simulink model "rfsoc4x2_ospfb_128"  (R2021a)
settings: Solver=VariableStepAuto  StartTime=0.0  StopTime=2048  RelTol=1e-3
undefined symbols (not defined in the file): pfb_coeff_gen_calc
libraries: xbsIndex_r4 x37092, casper_library_delays x737, casper_library_misc x68, xps_library x1
(part 120 of 339)

== system rfsoc4x2_ospfb_128/pfb_fir_real8/pol1_in9_last_tap ==
  din : Inport
  sync : Inport  Port=2
  coeff : Inport  Port=3
  Delay : xbsIndex_r4/Delay  rst=off  infoeditControl=Selection of Reset will increase slice count due to use of real FFs and instead of SRLs  en=off  latency=mult_latency  reg_retiming=off  dbl_ovrd=off  block_type=delay
      settings: xl_area=[0, 0, 0, 0, 0, 0, 0]  block_version=9.1.01
  Mult : xbsIndex_r4/Mult  precision=Full  arith_type="Signed  (2's comp)"  n_bits=8  bin_pt=2  quantization=Truncate  overflow=Wrap  en=off  latency=mult_latency  use_behavioral_HDL=on  opt=Speed  use_embedded=off  optimum_pipeline=off  pipeline=on  dbl_ovrd=off  use_rpm=on  placement_style=Rectangular shape  block_type=mult
      settings: infoedit=Hardware notes: To use the internal pipeline stage of the dedicated multiplier you must select 'Pipeline for maximum performance'.  xl_area=[0, 0, 0, 0, 0, 0, 0]  block_version=9.1.01
  Reinterpret : xbsIndex_r4/Reinterpret  force_arith_type=on  arith_type="Signed  (2's comp)"  force_bin_pt=on  bin_pt=CoeffBitWidth - 1  block_type=reinterpret
      settings: infoedit="Changes signal type without altering the binary representation.   You can changed the signal between signed and unsigned, and relocate the binary point.<P><P>Hardware notes: In hardware this block costs nothing.<P><P>Example:  Suppose the input is 6 bits wide, signed, with 2 fractional bits, and the output is forced to unsigned with 0 fractional bits.  Then an input of -2.0 (1110.00 in binary 2's complement) becomes an output of 56 (111000 in binary)."  block_version=9.1.01
  Reinterpret1 : xbsIndex_r4/Reinterpret  force_arith_type=on  arith_type="Signed  (2's comp)"  force_bin_pt=on  bin_pt=BitWidthIn - 1  block_type=reinterpret
      settings: infoedit="Changes signal type without altering the binary representation.   You can changed the signal between signed and unsigned, and relocate the binary point.<P><P>Hardware notes: In hardware this block costs nothing.<P><P>Example:  Suppose the input is 6 bits wide, signed, with 2 fractional bits, and the output is forced to unsigned with 0 fractional bits.  Then an input of -2.0 (1110.00 in binary 2's complement) becomes an output of 56 (111000 in binary)."  block_version=9.1.01
  tap_out : Outport  VectorParamsAs1DForOutWhenUnconnected=off
  sync_out : Outport  Port=2  VectorParamsAs1DForOutWhenUnconnected=off
  wires:
  Delay/1 -> sync_out/1
  din/1 -> Reinterpret1/1
  sync/1 -> Delay/1
  coeff/1 -> Reinterpret/1
  Reinterpret/1 -> Mult/2
  Mult/1 -> tap_out/1
  Reinterpret1/1 -> Mult/1

== system rfsoc4x2_ospfb_128/pfb_fir_real8/pol1_in9_tap2 ==
  din : Inport
  sync : Inport  Port=2
  coeff : Inport  Port=3
  Mult : xbsIndex_r4/Mult  precision=Full  arith_type="Signed  (2's comp)"  n_bits=8  bin_pt=2  quantization=Truncate  overflow=Wrap  en=off  latency=mult_latency  use_behavioral_HDL=on  opt=Speed  use_embedded=off  optimum_pipeline=off  pipeline=on  dbl_ovrd=off  use_rpm=on  placement_style=Rectangular shape  block_type=mult
      settings: infoedit=Hardware notes: To use the internal pipeline stage of the dedicated multiplier you must select 'Pipeline for maximum performance'.  xl_area=[0, 0, 0, 0, 0, 0, 0]  block_version=9.1.01
  Reinterpret : xbsIndex_r4/Reinterpret  force_arith_type=on  arith_type="Signed  (2's comp)"  force_bin_pt=on  bin_pt=coeff_frac_width  block_type=reinterpret
      settings: infoedit="Changes signal type without altering the binary representation.   You can changed the signal between signed and unsigned, and relocate the binary point.<P><P>Hardware notes: In hardware this block costs nothing.<P><P>Example:  Suppose the input is 6 bits wide, signed, with 2 fractional bits, and the output is forced to unsigned with 0 fractional bits.  Then an input of -2.0 (1110.00 in binary 2's complement) becomes an output of 56 (111000 in binary)."  block_version=9.1.01
  Reinterpret1 : xbsIndex_r4/Reinterpret  force_arith_type=on  arith_type="Signed  (2's comp)"  force_bin_pt=on  bin_pt=data_width - 1  block_type=reinterpret
      settings: infoedit="Changes signal type without altering the binary representation.   You can changed the signal between signed and unsigned, and relocate the binary point.<P><P>Hardware notes: In hardware this block costs nothing.<P><P>Example:  Suppose the input is 6 bits wide, signed, with 2 fractional bits, and the output is forced to unsigned with 0 fractional bits.  Then an input of -2.0 (1110.00 in binary 2's complement) becomes an output of 56 (111000 in binary)."  block_version=9.1.01
  Slice : xbsIndex_r4/Slice  nbits=coeff_width  boolean_output=off  mode=Lower Bit Location + Width  bit1=0  base1=MSB of Input  bit0=0  base0=LSB of Input  dbl_ovrd=off  block_type=slice
      settings: infoedit="Extracts a given range of bits from each input sample and presents it at the output.  The output type is ordinarily unsigned with binary point at zero, but can be Boolean when the slice is one bit wide.<P><P>Hardware notes: In hardware this block costs nothing."  block_version=9.1.01
  Slice1 : xbsIndex_r4/Slice  nbits=0  boolean_output=off  mode=Two Bit Locations  bit1=0  base1=MSB of Input  bit0=coeff_width  base0=LSB of Input  dbl_ovrd=off  block_type=slice
      settings: infoedit="Extracts a given range of bits from each input sample and presents it at the output.  The output type is ordinarily unsigned with binary point at zero, but can be Boolean when the slice is one bit wide.<P><P>Hardware notes: In hardware this block costs nothing."  block_version=9.1.01
  delay_bram : casper_library_delays/delay_bram  DelayLen=delay  bram_latency=bram_latency  use_dsp48=off  async=off
      settings: SourceProductName=CASPER DSP Blockset
  sync_delay : casper_library_delays/sync_delay  DelayLen=delay
      settings: SourceProductName=CASPER DSP Blockset
  dout : Outport  VectorParamsAs1DForOutWhenUnconnected=off
  sync_out : Outport  Port=2  VectorParamsAs1DForOutWhenUnconnected=off
  coeff_out : Outport  Port=3  VectorParamsAs1DForOutWhenUnconnected=off
  taps_out : Outport  Port=4  VectorParamsAs1DForOutWhenUnconnected=off
  wires:
  delay_bram/1 -> dout/1
  din/1 -> Reinterpret1/1, delay_bram/1
  Mult/1 -> taps_out/1
  sync/1 -> sync_delay/1
  sync_delay/1 -> sync_out/1
  coeff/1 -> Slice/1, Slice1/1
  Slice1/1 -> coeff_out/1
  Slice/1 -> Reinterpret/1
  Reinterpret/1 -> Mult/2
  Reinterpret1/1 -> Mult/1

== system rfsoc4x2_ospfb_128/pfb_fir_real8/pol1_in9_tap3 ==
  din : Inport
  sync : Inport  Port=2
  coeff : Inport  Port=3
  Mult : xbsIndex_r4/Mult  precision=Full  arith_type="Signed  (2's comp)"  n_bits=8  bin_pt=2  quantization=Truncate  overflow=Wrap  en=off  latency=mult_latency  use_behavioral_HDL=on  opt=Speed  use_embedded=off  optimum_pipeline=off  pipeline=on  dbl_ovrd=off  use_rpm=on  placement_style=Rectangular shape  block_type=mult
      settings: infoedit=Hardware notes: To use the internal pipeline stage of the dedicated multiplier you must select 'Pipeline for maximum performance'.  xl_area=[0, 0, 0, 0, 0, 0, 0]  block_version=9.1.01
  Reinterpret : xbsIndex_r4/Reinterpret  force_arith_type=on  arith_type="Signed  (2's comp)"  force_bin_pt=on  bin_pt=coeff_frac_width  block_type=reinterpret
      settings: infoedit="Changes signal type without altering the binary representation.   You can changed the signal between signed and unsigned, and relocate the binary point.<P><P>Hardware notes: In hardware this block costs nothing.<P><P>Example:  Suppose the input is 6 bits wide, signed, with 2 fractional bits, and the output is forced to unsigned with 0 fractional bits.  Then an input of -2.0 (1110.00 in binary 2's complement) becomes an output of 56 (111000 in binary)."  block_version=9.1.01
  Reinterpret1 : xbsIndex_r4/Reinterpret  force_arith_type=on  arith_type="Signed  (2's comp)"  force_bin_pt=on  bin_pt=data_width - 1  block_type=reinterpret
      settings: infoedit="Changes signal type without altering the binary representation.   You can changed the signal between signed and unsigned, and relocate the binary point.<P><P>Hardware notes: In hardware this block costs nothing.<P><P>Example:  Suppose the input is 6 bits wide, signed, with 2 fractional bits, and the output is forced to unsigned with 0 fractional bits.  Then an input of -2.0 (1110.00 in binary 2's complement) becomes an output of 56 (111000 in binary)."  block_version=9.1.01
  Slice : xbsIndex_r4/Slice  nbits=coeff_width  boolean_output=off  mode=Lower Bit Location + Width  bit1=0  base1=MSB of Input  bit0=0  base0=LSB of Input  dbl_ovrd=off  block_type=slice
      settings: infoedit="Extracts a given range of bits from each input sample and presents it at the output.  The output type is ordinarily unsigned with binary point at zero, but can be Boolean when the slice is one bit wide.<P><P>Hardware notes: In hardware this block costs nothing."  block_version=9.1.01
  Slice1 : xbsIndex_r4/Slice  nbits=0  boolean_output=off  mode=Two Bit Locations  bit1=0  base1=MSB of Input  bit0=coeff_width  base0=LSB of Input  dbl_ovrd=off  block_type=slice
      settings: infoedit="Extracts a given range of bits from each input sample and presents it at the output.  The output type is ordinarily unsigned with binary point at zero, but can be Boolean when the slice is one bit wide.<P><P>Hardware notes: In hardware this block costs nothing."  block_version=9.1.01
  delay_bram : casper_library_delays/delay_bram  DelayLen=delay  bram_latency=bram_latency  use_dsp48=off  async=off
      settings: SourceProductName=CASPER DSP Blockset
  sync_delay : casper_library_delays/sync_delay  DelayLen=delay
      settings: SourceProductName=CASPER DSP Blockset
  dout : Outport  VectorParamsAs1DForOutWhenUnconnected=off
  sync_out : Outport  Port=2  VectorParamsAs1DForOutWhenUnconnected=off
  coeff_out : Outport  Port=3  VectorParamsAs1DForOutWhenUnconnected=off
  taps_out : Outport  Port=4  VectorParamsAs1DForOutWhenUnconnected=off
  wires:
  delay_bram/1 -> dout/1
  din/1 -> Reinterpret1/1, delay_bram/1
  Mult/1 -> taps_out/1
  sync/1 -> sync_delay/1
  sync_delay/1 -> sync_out/1
  coeff/1 -> Slice/1, Slice1/1
  Slice1/1 -> coeff_out/1
  Slice/1 -> Reinterpret/1
  Reinterpret/1 -> Mult/2
  Reinterpret1/1 -> Mult/1

== system rfsoc4x2_ospfb_128/pfb_fir_real9/adder_1_1 ==
  sync : Inport
  din1 : Inport  Port=2
  din2 : Inport  Port=3
  din3 : Inport  Port=4
  din4 : Inport  Port=5
  din5 : Inport  Port=6
  din6 : Inport  Port=7
  din7 : Inport  Port=8
  din8 : Inport  Port=9
  addr{1..4} (4 alike) : xbsIndex_r4/AddSub  mode=Addition  use_carryin=off  use_carryout=off  en=off  latency=1  precision=User Defined  arith_type="Signed  (2's comp)"  n_bits=32  bin_pt=30  quantization=Truncate  overflow=Wrap  use_behavioral_HDL=on  hw_selection=Fabric  pipelined=on  use_rpm=on  dbl_ovrd=off  block_type=addsub
  addr5 : xbsIndex_r4/AddSub  mode=Addition  use_carryin=off  use_carryout=off  en=off  latency=1  precision=User Defined  arith_type="Signed  (2's comp)"  n_bits=32  bin_pt=30  quantization=Truncate  overflow=Wrap  use_behavioral_HDL=off  hw_selection=Fabric  pipelined=on  use_rpm=on  dbl_ovrd=off  block_type=addsub
  addr6 : xbsIndex_r4/AddSub  mode=Addition  use_carryin=off  use_carryout=off  en=off  latency=1  precision=User Defined  arith_type="Signed  (2's comp)"  n_bits=32  bin_pt=30  quantization=Truncate  overflow=Wrap  use_behavioral_HDL=off  hw_selection=Fabric  pipelined=on  use_rpm=on  dbl_ovrd=off  block_type=addsub
  addr7 : xbsIndex_r4/AddSub  mode=Addition  use_carryin=off  use_carryout=off  en=off  latency=1  precision=User Defined  arith_type="Signed  (2's comp)"  n_bits=32  bin_pt=30  quantization=Truncate  overflow=Wrap  use_behavioral_HDL=off  hw_selection=Fabric  pipelined=on  use_rpm=on  dbl_ovrd=off  block_type=addsub
  sync_delay : xbsIndex_r4/Delay  rst=off  infoeditControl=Selection of Reset will increase slice count due to use of real FFs and instead of SRLs  en=off  latency=3  reg_retiming=on  dbl_ovrd=off  block_type=delay
      settings: block_version=11.4
  sync_out : Outport  VectorParamsAs1DForOutWhenUnconnected=off
  dout : Outport  Port=2  VectorParamsAs1DForOutWhenUnconnected=off
  wires:
  sync/1 -> sync_delay/1
  sync_delay/1 -> sync_out/1
  din1/1 -> addr1/1
  din2/1 -> addr1/2
  din3/1 -> addr2/1
  din4/1 -> addr2/2
  din5/1 -> addr3/1
  din6/1 -> addr3/2
  din7/1 -> addr4/1
  din8/1 -> addr4/2
  addr1/1 -> addr5/1
  addr2/1 -> addr5/2
  addr3/1 -> addr6/1
  addr4/1 -> addr6/2
  addr5/1 -> addr7/1
  addr6/1 -> addr7/2
  addr7/1 -> dout/1

== system rfsoc4x2_ospfb_128/pfb_fir_real9/adder_1_10 ==
  sync : Inport
  din1 : Inport  Port=2
  din2 : Inport  Port=3
  din3 : Inport  Port=4
  din4 : Inport  Port=5
  din5 : Inport  Port=6
  din6 : Inport  Port=7
  din7 : Inport  Port=8
  din8 : Inport  Port=9
  addr{1..4} (4 alike) : xbsIndex_r4/AddSub  mode=Addition  use_carryin=off  use_carryout=off  en=off  latency=1  precision=User Defined  arith_type="Signed  (2's comp)"  n_bits=32  bin_pt=30  quantization=Truncate  overflow=Wrap  use_behavioral_HDL=on  hw_selection=Fabric  pipelined=on  use_rpm=on  dbl_ovrd=off  block_type=addsub
  addr5 : xbsIndex_r4/AddSub  mode=Addition  use_carryin=off  use_carryout=off  en=off  latency=1  precision=User Defined  arith_type="Signed  (2's comp)"  n_bits=32  bin_pt=30  quantization=Truncate  overflow=Wrap  use_behavioral_HDL=off  hw_selection=Fabric  pipelined=on  use_rpm=on  dbl_ovrd=off  block_type=addsub
  addr6 : xbsIndex_r4/AddSub  mode=Addition  use_carryin=off  use_carryout=off  en=off  latency=1  precision=User Defined  arith_type="Signed  (2's comp)"  n_bits=32  bin_pt=30  quantization=Truncate  overflow=Wrap  use_behavioral_HDL=off  hw_selection=Fabric  pipelined=on  use_rpm=on  dbl_ovrd=off  block_type=addsub
  addr7 : xbsIndex_r4/AddSub  mode=Addition  use_carryin=off  use_carryout=off  en=off  latency=1  precision=User Defined  arith_type="Signed  (2's comp)"  n_bits=32  bin_pt=30  quantization=Truncate  overflow=Wrap  use_behavioral_HDL=off  hw_selection=Fabric  pipelined=on  use_rpm=on  dbl_ovrd=off  block_type=addsub
  sync_delay : xbsIndex_r4/Delay  rst=off  infoeditControl=Selection of Reset will increase slice count due to use of real FFs and instead of SRLs  en=off  latency=3  reg_retiming=on  dbl_ovrd=off  block_type=delay
      settings: block_version=11.4
  sync_out : Outport  VectorParamsAs1DForOutWhenUnconnected=off
  dout : Outport  Port=2  VectorParamsAs1DForOutWhenUnconnected=off
  wires:
  sync/1 -> sync_delay/1
  sync_delay/1 -> sync_out/1
  din1/1 -> addr1/1
  din2/1 -> addr1/2
  din3/1 -> addr2/1
  din4/1 -> addr2/2
  din5/1 -> addr3/1
  din6/1 -> addr3/2
  din7/1 -> addr4/1
  din8/1 -> addr4/2
  addr1/1 -> addr5/1
  addr2/1 -> addr5/2
  addr3/1 -> addr6/1
  addr4/1 -> addr6/2
  addr5/1 -> addr7/1
  addr6/1 -> addr7/2
  addr7/1 -> dout/1

== system rfsoc4x2_ospfb_128/pfb_fir_real9/adder_1_11 ==
  sync : Inport
  din1 : Inport  Port=2
  din2 : Inport  Port=3
  din3 : Inport  Port=4
  din4 : Inport  Port=5
  din5 : Inport  Port=6
  din6 : Inport  Port=7
  din7 : Inport  Port=8
  din8 : Inport  Port=9
  addr{1..4} (4 alike) : xbsIndex_r4/AddSub  mode=Addition  use_carryin=off  use_carryout=off  en=off  latency=1  precision=User Defined  arith_type="Signed  (2's comp)"  n_bits=32  bin_pt=30  quantization=Truncate  overflow=Wrap  use_behavioral_HDL=on  hw_selection=Fabric  pipelined=on  use_rpm=on  dbl_ovrd=off  block_type=addsub
  addr5 : xbsIndex_r4/AddSub  mode=Addition  use_carryin=off  use_carryout=off  en=off  latency=1  precision=User Defined  arith_type="Signed  (2's comp)"  n_bits=32  bin_pt=30  quantization=Truncate  overflow=Wrap  use_behavioral_HDL=off  hw_selection=Fabric  pipelined=on  use_rpm=on  dbl_ovrd=off  block_type=addsub
  addr6 : xbsIndex_r4/AddSub  mode=Addition  use_carryin=off  use_carryout=off  en=off  latency=1  precision=User Defined  arith_type="Signed  (2's comp)"  n_bits=32  bin_pt=30  quantization=Truncate  overflow=Wrap  use_behavioral_HDL=off  hw_selection=Fabric  pipelined=on  use_rpm=on  dbl_ovrd=off  block_type=addsub
  addr7 : xbsIndex_r4/AddSub  mode=Addition  use_carryin=off  use_carryout=off  en=off  latency=1  precision=User Defined  arith_type="Signed  (2's comp)"  n_bits=32  bin_pt=30  quantization=Truncate  overflow=Wrap  use_behavioral_HDL=off  hw_selection=Fabric  pipelined=on  use_rpm=on  dbl_ovrd=off  block_type=addsub
  sync_delay : xbsIndex_r4/Delay  rst=off  infoeditControl=Selection of Reset will increase slice count due to use of real FFs and instead of SRLs  en=off  latency=3  reg_retiming=on  dbl_ovrd=off  block_type=delay
      settings: block_version=11.4
  sync_out : Outport  VectorParamsAs1DForOutWhenUnconnected=off
  dout : Outport  Port=2  VectorParamsAs1DForOutWhenUnconnected=off
  wires:
  sync/1 -> sync_delay/1
  sync_delay/1 -> sync_out/1
  din1/1 -> addr1/1
  din2/1 -> addr1/2
  din3/1 -> addr2/1
  din4/1 -> addr2/2
  din5/1 -> addr3/1
  din6/1 -> addr3/2
  din7/1 -> addr4/1
  din8/1 -> addr4/2
  addr1/1 -> addr5/1
  addr2/1 -> addr5/2
  addr3/1 -> addr6/1
  addr4/1 -> addr6/2
  addr5/1 -> addr7/1
  addr6/1 -> addr7/2
  addr7/1 -> dout/1

== system rfsoc4x2_ospfb_128/pfb_fir_real9/adder_1_12 ==
  sync : Inport
  din1 : Inport  Port=2
  din2 : Inport  Port=3
  din3 : Inport  Port=4
  din4 : Inport  Port=5
  din5 : Inport  Port=6
  din6 : Inport  Port=7
  din7 : Inport  Port=8
  din8 : Inport  Port=9
  addr{1..4} (4 alike) : xbsIndex_r4/AddSub  mode=Addition  use_carryin=off  use_carryout=off  en=off  latency=1  precision=User Defined  arith_type="Signed  (2's comp)"  n_bits=32  bin_pt=30  quantization=Truncate  overflow=Wrap  use_behavioral_HDL=on  hw_selection=Fabric  pipelined=on  use_rpm=on  dbl_ovrd=off  block_type=addsub
  addr5 : xbsIndex_r4/AddSub  mode=Addition  use_carryin=off  use_carryout=off  en=off  latency=1  precision=User Defined  arith_type="Signed  (2's comp)"  n_bits=32  bin_pt=30  quantization=Truncate  overflow=Wrap  use_behavioral_HDL=off  hw_selection=Fabric  pipelined=on  use_rpm=on  dbl_ovrd=off  block_type=addsub
  addr6 : xbsIndex_r4/AddSub  mode=Addition  use_carryin=off  use_carryout=off  en=off  latency=1  precision=User Defined  arith_type="Signed  (2's comp)"  n_bits=32  bin_pt=30  quantization=Truncate  overflow=Wrap  use_behavioral_HDL=off  hw_selection=Fabric  pipelined=on  use_rpm=on  dbl_ovrd=off  block_type=addsub
  addr7 : xbsIndex_r4/AddSub  mode=Addition  use_carryin=off  use_carryout=off  en=off  latency=1  precision=User Defined  arith_type="Signed  (2's comp)"  n_bits=32  bin_pt=30  quantization=Truncate  overflow=Wrap  use_behavioral_HDL=off  hw_selection=Fabric  pipelined=on  use_rpm=on  dbl_ovrd=off  block_type=addsub
  sync_delay : xbsIndex_r4/Delay  rst=off  infoeditControl=Selection of Reset will increase slice count due to use of real FFs and instead of SRLs  en=off  latency=3  reg_retiming=on  dbl_ovrd=off  block_type=delay
      settings: block_version=11.4
  sync_out : Outport  VectorParamsAs1DForOutWhenUnconnected=off
  dout : Outport  Port=2  VectorParamsAs1DForOutWhenUnconnected=off
  wires:
  sync/1 -> sync_delay/1
  sync_delay/1 -> sync_out/1
  din1/1 -> addr1/1
  din2/1 -> addr1/2
  din3/1 -> addr2/1
  din4/1 -> addr2/2
  din5/1 -> addr3/1
  din6/1 -> addr3/2
  din7/1 -> addr4/1
  din8/1 -> addr4/2
  addr1/1 -> addr5/1
  addr2/1 -> addr5/2
  addr3/1 -> addr6/1
  addr4/1 -> addr6/2
  addr5/1 -> addr7/1
  addr6/1 -> addr7/2
  addr7/1 -> dout/1

== system rfsoc4x2_ospfb_128/pfb_fir_real9/adder_1_13 ==
  sync : Inport
  din1 : Inport  Port=2
  din2 : Inport  Port=3
  din3 : Inport  Port=4
  din4 : Inport  Port=5
  din5 : Inport  Port=6
  din6 : Inport  Port=7
  din7 : Inport  Port=8
  din8 : Inport  Port=9
  addr{1..4} (4 alike) : xbsIndex_r4/AddSub  mode=Addition  use_carryin=off  use_carryout=off  en=off  latency=1  precision=User Defined  arith_type="Signed  (2's comp)"  n_bits=32  bin_pt=30  quantization=Truncate  overflow=Wrap  use_behavioral_HDL=on  hw_selection=Fabric  pipelined=on  use_rpm=on  dbl_ovrd=off  block_type=addsub
  addr5 : xbsIndex_r4/AddSub  mode=Addition  use_carryin=off  use_carryout=off  en=off  latency=1  precision=User Defined  arith_type="Signed  (2's comp)"  n_bits=32  bin_pt=30  quantization=Truncate  overflow=Wrap  use_behavioral_HDL=off  hw_selection=Fabric  pipelined=on  use_rpm=on  dbl_ovrd=off  block_type=addsub
  addr6 : xbsIndex_r4/AddSub  mode=Addition  use_carryin=off  use_carryout=off  en=off  latency=1  precision=User Defined  arith_type="Signed  (2's comp)"  n_bits=32  bin_pt=30  quantization=Truncate  overflow=Wrap  use_behavioral_HDL=off  hw_selection=Fabric  pipelined=on  use_rpm=on  dbl_ovrd=off  block_type=addsub
  addr7 : xbsIndex_r4/AddSub  mode=Addition  use_carryin=off  use_carryout=off  en=off  latency=1  precision=User Defined  arith_type="Signed  (2's comp)"  n_bits=32  bin_pt=30  quantization=Truncate  overflow=Wrap  use_behavioral_HDL=off  hw_selection=Fabric  pipelined=on  use_rpm=on  dbl_ovrd=off  block_type=addsub
  sync_delay : xbsIndex_r4/Delay  rst=off  infoeditControl=Selection of Reset will increase slice count due to use of real FFs and instead of SRLs  en=off  latency=3  reg_retiming=on  dbl_ovrd=off  block_type=delay
      settings: block_version=11.4
  sync_out : Outport  VectorParamsAs1DForOutWhenUnconnected=off
  dout : Outport  Port=2  VectorParamsAs1DForOutWhenUnconnected=off
  wires:
  sync/1 -> sync_delay/1
  sync_delay/1 -> sync_out/1
  din1/1 -> addr1/1
  din2/1 -> addr1/2
  din3/1 -> addr2/1
  din4/1 -> addr2/2
  din5/1 -> addr3/1
  din6/1 -> addr3/2
  din7/1 -> addr4/1
  din8/1 -> addr4/2
  addr1/1 -> addr5/1
  addr2/1 -> addr5/2
  addr3/1 -> addr6/1
  addr4/1 -> addr6/2
  addr5/1 -> addr7/1
  addr6/1 -> addr7/2
  addr7/1 -> dout/1

== system rfsoc4x2_ospfb_128/pfb_fir_real9/adder_1_14 ==
  sync : Inport
  din1 : Inport  Port=2
  din2 : Inport  Port=3
  din3 : Inport  Port=4
  din4 : Inport  Port=5
  din5 : Inport  Port=6
  din6 : Inport  Port=7
  din7 : Inport  Port=8
  din8 : Inport  Port=9
  addr{1..4} (4 alike) : xbsIndex_r4/AddSub  mode=Addition  use_carryin=off  use_carryout=off  en=off  latency=1  precision=User Defined  arith_type="Signed  (2's comp)"  n_bits=32  bin_pt=30  quantization=Truncate  overflow=Wrap  use_behavioral_HDL=on  hw_selection=Fabric  pipelined=on  use_rpm=on  dbl_ovrd=off  block_type=addsub
  addr5 : xbsIndex_r4/AddSub  mode=Addition  use_carryin=off  use_carryout=off  en=off  latency=1  precision=User Defined  arith_type="Signed  (2's comp)"  n_bits=32  bin_pt=30  quantization=Truncate  overflow=Wrap  use_behavioral_HDL=off  hw_selection=Fabric  pipelined=on  use_rpm=on  dbl_ovrd=off  block_type=addsub
  addr6 : xbsIndex_r4/AddSub  mode=Addition  use_carryin=off  use_carryout=off  en=off  latency=1  precision=User Defined  arith_type="Signed  (2's comp)"  n_bits=32  bin_pt=30  quantization=Truncate  overflow=Wrap  use_behavioral_HDL=off  hw_selection=Fabric  pipelined=on  use_rpm=on  dbl_ovrd=off  block_type=addsub
  addr7 : xbsIndex_r4/AddSub  mode=Addition  use_carryin=off  use_carryout=off  en=off  latency=1  precision=User Defined  arith_type="Signed  (2's comp)"  n_bits=32  bin_pt=30  quantization=Truncate  overflow=Wrap  use_behavioral_HDL=off  hw_selection=Fabric  pipelined=on  use_rpm=on  dbl_ovrd=off  block_type=addsub
  sync_delay : xbsIndex_r4/Delay  rst=off  infoeditControl=Selection of Reset will increase slice count due to use of real FFs and instead of SRLs  en=off  latency=3  reg_retiming=on  dbl_ovrd=off  block_type=delay
      settings: block_version=11.4
  sync_out : Outport  VectorParamsAs1DForOutWhenUnconnected=off
  dout : Outport  Port=2  VectorParamsAs1DForOutWhenUnconnected=off
  wires:
  sync/1 -> sync_delay/1
  sync_delay/1 -> sync_out/1
  din1/1 -> addr1/1
  din2/1 -> addr1/2
  din3/1 -> addr2/1
  din4/1 -> addr2/2
  din5/1 -> addr3/1
  din6/1 -> addr3/2
  din7/1 -> addr4/1
  din8/1 -> addr4/2
  addr1/1 -> addr5/1
  addr2/1 -> addr5/2
  addr3/1 -> addr6/1
  addr4/1 -> addr6/2
  addr5/1 -> addr7/1
  addr6/1 -> addr7/2
  addr7/1 -> dout/1

== system rfsoc4x2_ospfb_128/pfb_fir_real9/adder_1_15 ==
  sync : Inport
  din1 : Inport  Port=2
  din2 : Inport  Port=3
  din3 : Inport  Port=4
  din4 : Inport  Port=5
  din5 : Inport  Port=6
  din6 : Inport  Port=7
  din7 : Inport  Port=8
  din8 : Inport  Port=9
  addr{1..4} (4 alike) : xbsIndex_r4/AddSub  mode=Addition  use_carryin=off  use_carryout=off  en=off  latency=1  precision=User Defined  arith_type="Signed  (2's comp)"  n_bits=32  bin_pt=30  quantization=Truncate  overflow=Wrap  use_behavioral_HDL=on  hw_selection=Fabric  pipelined=on  use_rpm=on  dbl_ovrd=off  block_type=addsub
  addr5 : xbsIndex_r4/AddSub  mode=Addition  use_carryin=off  use_carryout=off  en=off  latency=1  precision=User Defined  arith_type="Signed  (2's comp)"  n_bits=32  bin_pt=30  quantization=Truncate  overflow=Wrap  use_behavioral_HDL=off  hw_selection=Fabric  pipelined=on  use_rpm=on  dbl_ovrd=off  block_type=addsub
  addr6 : xbsIndex_r4/AddSub  mode=Addition  use_carryin=off  use_carryout=off  en=off  latency=1  precision=User Defined  arith_type="Signed  (2's comp)"  n_bits=32  bin_pt=30  quantization=Truncate  overflow=Wrap  use_behavioral_HDL=off  hw_selection=Fabric  pipelined=on  use_rpm=on  dbl_ovrd=off  block_type=addsub
  addr7 : xbsIndex_r4/AddSub  mode=Addition  use_carryin=off  use_carryout=off  en=off  latency=1  precision=User Defined  arith_type="Signed  (2's comp)"  n_bits=32  bin_pt=30  quantization=Truncate  overflow=Wrap  use_behavioral_HDL=off  hw_selection=Fabric  pipelined=on  use_rpm=on  dbl_ovrd=off  block_type=addsub
  sync_delay : xbsIndex_r4/Delay  rst=off  infoeditControl=Selection of Reset will increase slice count due to use of real FFs and instead of SRLs  en=off  latency=3  reg_retiming=on  dbl_ovrd=off  block_type=delay
      settings: block_version=11.4
  sync_out : Outport  VectorParamsAs1DForOutWhenUnconnected=off
  dout : Outport  Port=2  VectorParamsAs1DForOutWhenUnconnected=off
  wires:
  sync/1 -> sync_delay/1
  sync_delay/1 -> sync_out/1
  din1/1 -> addr1/1
  din2/1 -> addr1/2
  din3/1 -> addr2/1
  din4/1 -> addr2/2
  din5/1 -> addr3/1
  din6/1 -> addr3/2
  din7/1 -> addr4/1
  din8/1 -> addr4/2
  addr1/1 -> addr5/1
  addr2/1 -> addr5/2
  addr3/1 -> addr6/1
  addr4/1 -> addr6/2
  addr5/1 -> addr7/1
  addr6/1 -> addr7/2
  addr7/1 -> dout/1

== system rfsoc4x2_ospfb_128/pfb_fir_real9/adder_1_16 ==
  sync : Inport
  din1 : Inport  Port=2
  din2 : Inport  Port=3
  din3 : Inport  Port=4
  din4 : Inport  Port=5
  din5 : Inport  Port=6
  din6 : Inport  Port=7
  din7 : Inport  Port=8
  din8 : Inport  Port=9
  addr{1..4} (4 alike) : xbsIndex_r4/AddSub  mode=Addition  use_carryin=off  use_carryout=off  en=off  latency=1  precision=User Defined  arith_type="Signed  (2's comp)"  n_bits=32  bin_pt=30  quantization=Truncate  overflow=Wrap  use_behavioral_HDL=on  hw_selection=Fabric  pipelined=on  use_rpm=on  dbl_ovrd=off  block_type=addsub
  addr5 : xbsIndex_r4/AddSub  mode=Addition  use_carryin=off  use_carryout=off  en=off  latency=1  precision=User Defined  arith_type="Signed  (2's comp)"  n_bits=32  bin_pt=30  quantization=Truncate  overflow=Wrap  use_behavioral_HDL=off  hw_selection=Fabric  pipelined=on  use_rpm=on  dbl_ovrd=off  block_type=addsub
  addr6 : xbsIndex_r4/AddSub  mode=Addition  use_carryin=off  use_carryout=off  en=off  latency=1  precision=User Defined  arith_type="Signed  (2's comp)"  n_bits=32  bin_pt=30  quantization=Truncate  overflow=Wrap  use_behavioral_HDL=off  hw_selection=Fabric  pipelined=on  use_rpm=on  dbl_ovrd=off  block_type=addsub
  addr7 : xbsIndex_r4/AddSub  mode=Addition  use_carryin=off  use_carryout=off  en=off  latency=1  precision=User Defined  arith_type="Signed  (2's comp)"  n_bits=32  bin_pt=30  quantization=Truncate  overflow=Wrap  use_behavioral_HDL=off  hw_selection=Fabric  pipelined=on  use_rpm=on  dbl_ovrd=off  block_type=addsub
  sync_delay : xbsIndex_r4/Delay  rst=off  infoeditControl=Selection of Reset will increase slice count due to use of real FFs and instead of SRLs  en=off  latency=3  reg_retiming=on  dbl_ovrd=off  block_type=delay
      settings: block_version=11.4
  sync_out : Outport  VectorParamsAs1DForOutWhenUnconnected=off
  dout : Outport  Port=2  VectorParamsAs1DForOutWhenUnconnected=off
  wires:
  sync/1 -> sync_delay/1
  sync_delay/1 -> sync_out/1
  din1/1 -> addr1/1
  din2/1 -> addr1/2
  din3/1 -> addr2/1
  din4/1 -> addr2/2
  din5/1 -> addr3/1
  din6/1 -> addr3/2
  din7/1 -> addr4/1
  din8/1 -> addr4/2
  addr1/1 -> addr5/1
  addr2/1 -> addr5/2
  addr3/1 -> addr6/1
  addr4/1 -> addr6/2
  addr5/1 -> addr7/1
  addr6/1 -> addr7/2
  addr7/1 -> dout/1

== system rfsoc4x2_ospfb_128/pfb_fir_real9/adder_1_2 ==
  sync : Inport
  din1 : Inport  Port=2
  din2 : Inport  Port=3
  din3 : Inport  Port=4
  din4 : Inport  Port=5
  din5 : Inport  Port=6
  din6 : Inport  Port=7
  din7 : Inport  Port=8
  din8 : Inport  Port=9
  addr{1..4} (4 alike) : xbsIndex_r4/AddSub  mode=Addition  use_carryin=off  use_carryout=off  en=off  latency=1  precision=User Defined  arith_type="Signed  (2's comp)"  n_bits=32  bin_pt=30  quantization=Truncate  overflow=Wrap  use_behavioral_HDL=on  hw_selection=Fabric  pipelined=on  use_rpm=on  dbl_ovrd=off  block_type=addsub
  addr5 : xbsIndex_r4/AddSub  mode=Addition  use_carryin=off  use_carryout=off  en=off  latency=1  precision=User Defined  arith_type="Signed  (2's comp)"  n_bits=32  bin_pt=30  quantization=Truncate  overflow=Wrap  use_behavioral_HDL=off  hw_selection=Fabric  pipelined=on  use_rpm=on  dbl_ovrd=off  block_type=addsub
  addr6 : xbsIndex_r4/AddSub  mode=Addition  use_carryin=off  use_carryout=off  en=off  latency=1  precision=User Defined  arith_type="Signed  (2's comp)"  n_bits=32  bin_pt=30  quantization=Truncate  overflow=Wrap  use_behavioral_HDL=off  hw_selection=Fabric  pipelined=on  use_rpm=on  dbl_ovrd=off  block_type=addsub
  addr7 : xbsIndex_r4/AddSub  mode=Addition  use_carryin=off  use_carryout=off  en=off  latency=1  precision=User Defined  arith_type="Signed  (2's comp)"  n_bits=32  bin_pt=30  quantization=Truncate  overflow=Wrap  use_behavioral_HDL=off  hw_selection=Fabric  pipelined=on  use_rpm=on  dbl_ovrd=off  block_type=addsub
  sync_delay : xbsIndex_r4/Delay  rst=off  infoeditControl=Selection of Reset will increase slice count due to use of real FFs and instead of SRLs  en=off  latency=3  reg_retiming=on  dbl_ovrd=off  block_type=delay
      settings: block_version=11.4
  sync_out : Outport  VectorParamsAs1DForOutWhenUnconnected=off
  dout : Outport  Port=2  VectorParamsAs1DForOutWhenUnconnected=off
  wires:
  sync/1 -> sync_delay/1
  sync_delay/1 -> sync_out/1
  din1/1 -> addr1/1
  din2/1 -> addr1/2
  din3/1 -> addr2/1
  din4/1 -> addr2/2
  din5/1 -> addr3/1
  din6/1 -> addr3/2
  din7/1 -> addr4/1
  din8/1 -> addr4/2
  addr1/1 -> addr5/1
  addr2/1 -> addr5/2
  addr3/1 -> addr6/1
  addr4/1 -> addr6/2
  addr5/1 -> addr7/1
  addr6/1 -> addr7/2
  addr7/1 -> dout/1

== system rfsoc4x2_ospfb_128/pfb_fir_real9/adder_1_3 ==
  sync : Inport
  din1 : Inport  Port=2
  din2 : Inport  Port=3
  din3 : Inport  Port=4
  din4 : Inport  Port=5
  din5 : Inport  Port=6
  din6 : Inport  Port=7
  din7 : Inport  Port=8
  din8 : Inport  Port=9
  addr{1..4} (4 alike) : xbsIndex_r4/AddSub  mode=Addition  use_carryin=off  use_carryout=off  en=off  latency=1  precision=User Defined  arith_type="Signed  (2's comp)"  n_bits=32  bin_pt=30  quantization=Truncate  overflow=Wrap  use_behavioral_HDL=on  hw_selection=Fabric  pipelined=on  use_rpm=on  dbl_ovrd=off  block_type=addsub
  addr5 : xbsIndex_r4/AddSub  mode=Addition  use_carryin=off  use_carryout=off  en=off  latency=1  precision=User Defined  arith_type="Signed  (2's comp)"  n_bits=32  bin_pt=30  quantization=Truncate  overflow=Wrap  use_behavioral_HDL=off  hw_selection=Fabric  pipelined=on  use_rpm=on  dbl_ovrd=off  block_type=addsub
  addr6 : xbsIndex_r4/AddSub  mode=Addition  use_carryin=off  use_carryout=off  en=off  latency=1  precision=User Defined  arith_type="Signed  (2's comp)"  n_bits=32  bin_pt=30  quantization=Truncate  overflow=Wrap  use_behavioral_HDL=off  hw_selection=Fabric  pipelined=on  use_rpm=on  dbl_ovrd=off  block_type=addsub
  addr7 : xbsIndex_r4/AddSub  mode=Addition  use_carryin=off  use_carryout=off  en=off  latency=1  precision=User Defined  arith_type="Signed  (2's comp)"  n_bits=32  bin_pt=30  quantization=Truncate  overflow=Wrap  use_behavioral_HDL=off  hw_selection=Fabric  pipelined=on  use_rpm=on  dbl_ovrd=off  block_type=addsub
  sync_delay : xbsIndex_r4/Delay  rst=off  infoeditControl=Selection of Reset will increase slice count due to use of real FFs and instead of SRLs  en=off  latency=3  reg_retiming=on  dbl_ovrd=off  block_type=delay
      settings: block_version=11.4
  sync_out : Outport  VectorParamsAs1DForOutWhenUnconnected=off
  dout : Outport  Port=2  VectorParamsAs1DForOutWhenUnconnected=off
  wires:
  sync/1 -> sync_delay/1
  sync_delay/1 -> sync_out/1
  din1/1 -> addr1/1
  din2/1 -> addr1/2
  din3/1 -> addr2/1
  din4/1 -> addr2/2
  din5/1 -> addr3/1
  din6/1 -> addr3/2
  din7/1 -> addr4/1
  din8/1 -> addr4/2
  addr1/1 -> addr5/1
  addr2/1 -> addr5/2
  addr3/1 -> addr6/1
  addr4/1 -> addr6/2
  addr5/1 -> addr7/1
  addr6/1 -> addr7/2
  addr7/1 -> dout/1

== system rfsoc4x2_ospfb_128/pfb_fir_real9/adder_1_4 ==
  sync : Inport
  din1 : Inport  Port=2
  din2 : Inport  Port=3
  din3 : Inport  Port=4
  din4 : Inport  Port=5
  din5 : Inport  Port=6
  din6 : Inport  Port=7
  din7 : Inport  Port=8
  din8 : Inport  Port=9
  addr{1..4} (4 alike) : xbsIndex_r4/AddSub  mode=Addition  use_carryin=off  use_carryout=off  en=off  latency=1  precision=User Defined  arith_type="Signed  (2's comp)"  n_bits=32  bin_pt=30  quantization=Truncate  overflow=Wrap  use_behavioral_HDL=on  hw_selection=Fabric  pipelined=on  use_rpm=on  dbl_ovrd=off  block_type=addsub
  addr5 : xbsIndex_r4/AddSub  mode=Addition  use_carryin=off  use_carryout=off  en=off  latency=1  precision=User Defined  arith_type="Signed  (2's comp)"  n_bits=32  bin_pt=30  quantization=Truncate  overflow=Wrap  use_behavioral_HDL=off  hw_selection=Fabric  pipelined=on  use_rpm=on  dbl_ovrd=off  block_type=addsub
  addr6 : xbsIndex_r4/AddSub  mode=Addition  use_carryin=off  use_carryout=off  en=off  latency=1  precision=User Defined  arith_type="Signed  (2's comp)"  n_bits=32  bin_pt=30  quantization=Truncate  overflow=Wrap  use_behavioral_HDL=off  hw_selection=Fabric  pipelined=on  use_rpm=on  dbl_ovrd=off  block_type=addsub
  addr7 : xbsIndex_r4/AddSub  mode=Addition  use_carryin=off  use_carryout=off  en=off  latency=1  precision=User Defined  arith_type="Signed  (2's comp)"  n_bits=32  bin_pt=30  quantization=Truncate  overflow=Wrap  use_behavioral_HDL=off  hw_selection=Fabric  pipelined=on  use_rpm=on  dbl_ovrd=off  block_type=addsub
  sync_delay : xbsIndex_r4/Delay  rst=off  infoeditControl=Selection of Reset will increase slice count due to use of real FFs and instead of SRLs  en=off  latency=3  reg_retiming=on  dbl_ovrd=off  block_type=delay
      settings: block_version=11.4
  sync_out : Outport  VectorParamsAs1DForOutWhenUnconnected=off
  dout : Outport  Port=2  VectorParamsAs1DForOutWhenUnconnected=off
  wires:
  sync/1 -> sync_delay/1
  sync_delay/1 -> sync_out/1
  din1/1 -> addr1/1
  din2/1 -> addr1/2
  din3/1 -> addr2/1
  din4/1 -> addr2/2
  din5/1 -> addr3/1
  din6/1 -> addr3/2
  din7/1 -> addr4/1
  din8/1 -> addr4/2
  addr1/1 -> addr5/1
  addr2/1 -> addr5/2
  addr3/1 -> addr6/1
  addr4/1 -> addr6/2
  addr5/1 -> addr7/1
  addr6/1 -> addr7/2
  addr7/1 -> dout/1

== system rfsoc4x2_ospfb_128/pfb_fir_real9/adder_1_5 ==
  sync : Inport
  din1 : Inport  Port=2
  din2 : Inport  Port=3
  din3 : Inport  Port=4
  din4 : Inport  Port=5
  din5 : Inport  Port=6
  din6 : Inport  Port=7
  din7 : Inport  Port=8
  din8 : Inport  Port=9
  addr{1..4} (4 alike) : xbsIndex_r4/AddSub  mode=Addition  use_carryin=off  use_carryout=off  en=off  latency=1  precision=User Defined  arith_type="Signed  (2's comp)"  n_bits=32  bin_pt=30  quantization=Truncate  overflow=Wrap  use_behavioral_HDL=on  hw_selection=Fabric  pipelined=on  use_rpm=on  dbl_ovrd=off  block_type=addsub
  addr5 : xbsIndex_r4/AddSub  mode=Addition  use_carryin=off  use_carryout=off  en=off  latency=1  precision=User Defined  arith_type="Signed  (2's comp)"  n_bits=32  bin_pt=30  quantization=Truncate  overflow=Wrap  use_behavioral_HDL=off  hw_selection=Fabric  pipelined=on  use_rpm=on  dbl_ovrd=off  block_type=addsub
  addr6 : xbsIndex_r4/AddSub  mode=Addition  use_carryin=off  use_carryout=off  en=off  latency=1  precision=User Defined  arith_type="Signed  (2's comp)"  n_bits=32  bin_pt=30  quantization=Truncate  overflow=Wrap  use_behavioral_HDL=off  hw_selection=Fabric  pipelined=on  use_rpm=on  dbl_ovrd=off  block_type=addsub
  addr7 : xbsIndex_r4/AddSub  mode=Addition  use_carryin=off  use_carryout=off  en=off  latency=1  precision=User Defined  arith_type="Signed  (2's comp)"  n_bits=32  bin_pt=30  quantization=Truncate  overflow=Wrap  use_behavioral_HDL=off  hw_selection=Fabric  pipelined=on  use_rpm=on  dbl_ovrd=off  block_type=addsub
  sync_delay : xbsIndex_r4/Delay  rst=off  infoeditControl=Selection of Reset will increase slice count due to use of real FFs and instead of SRLs  en=off  latency=3  reg_retiming=on  dbl_ovrd=off  block_type=delay
      settings: block_version=11.4
  sync_out : Outport  VectorParamsAs1DForOutWhenUnconnected=off
  dout : Outport  Port=2  VectorParamsAs1DForOutWhenUnconnected=off
  wires:
  sync/1 -> sync_delay/1
  sync_delay/1 -> sync_out/1
  din1/1 -> addr1/1
  din2/1 -> addr1/2
  din3/1 -> addr2/1
  din4/1 -> addr2/2
  din5/1 -> addr3/1
  din6/1 -> addr3/2
  din7/1 -> addr4/1
  din8/1 -> addr4/2
  addr1/1 -> addr5/1
  addr2/1 -> addr5/2
  addr3/1 -> addr6/1
  addr4/1 -> addr6/2
  addr5/1 -> addr7/1
  addr6/1 -> addr7/2
  addr7/1 -> dout/1

== system rfsoc4x2_ospfb_128/pfb_fir_real9/adder_1_6 ==
  sync : Inport
  din1 : Inport  Port=2
  din2 : Inport  Port=3
  din3 : Inport  Port=4
  din4 : Inport  Port=5
  din5 : Inport  Port=6
  din6 : Inport  Port=7
  din7 : Inport  Port=8
  din8 : Inport  Port=9
  addr{1..4} (4 alike) : xbsIndex_r4/AddSub  mode=Addition  use_carryin=off  use_carryout=off  en=off  latency=1  precision=User Defined  arith_type="Signed  (2's comp)"  n_bits=32  bin_pt=30  quantization=Truncate  overflow=Wrap  use_behavioral_HDL=on  hw_selection=Fabric  pipelined=on  use_rpm=on  dbl_ovrd=off  block_type=addsub
  addr5 : xbsIndex_r4/AddSub  mode=Addition  use_carryin=off  use_carryout=off  en=off  latency=1  precision=User Defined  arith_type="Signed  (2's comp)"  n_bits=32  bin_pt=30  quantization=Truncate  overflow=Wrap  use_behavioral_HDL=off  hw_selection=Fabric  pipelined=on  use_rpm=on  dbl_ovrd=off  block_type=addsub
  addr6 : xbsIndex_r4/AddSub  mode=Addition  use_carryin=off  use_carryout=off  en=off  latency=1  precision=User Defined  arith_type="Signed  (2's comp)"  n_bits=32  bin_pt=30  quantization=Truncate  overflow=Wrap  use_behavioral_HDL=off  hw_selection=Fabric  pipelined=on  use_rpm=on  dbl_ovrd=off  block_type=addsub
  addr7 : xbsIndex_r4/AddSub  mode=Addition  use_carryin=off  use_carryout=off  en=off  latency=1  precision=User Defined  arith_type="Signed  (2's comp)"  n_bits=32  bin_pt=30  quantization=Truncate  overflow=Wrap  use_behavioral_HDL=off  hw_selection=Fabric  pipelined=on  use_rpm=on  dbl_ovrd=off  block_type=addsub
  sync_delay : xbsIndex_r4/Delay  rst=off  infoeditControl=Selection of Reset will increase slice count due to use of real FFs and instead of SRLs  en=off  latency=3  reg_retiming=on  dbl_ovrd=off  block_type=delay
      settings: block_version=11.4
  sync_out : Outport  VectorParamsAs1DForOutWhenUnconnected=off
  dout : Outport  Port=2  VectorParamsAs1DForOutWhenUnconnected=off
  wires:
  sync/1 -> sync_delay/1
  sync_delay/1 -> sync_out/1
  din1/1 -> addr1/1
  din2/1 -> addr1/2
  din3/1 -> addr2/1
  din4/1 -> addr2/2
  din5/1 -> addr3/1
  din6/1 -> addr3/2
  din7/1 -> addr4/1
  din8/1 -> addr4/2
  addr1/1 -> addr5/1
  addr2/1 -> addr5/2
  addr3/1 -> addr6/1
  addr4/1 -> addr6/2
  addr5/1 -> addr7/1
  addr6/1 -> addr7/2
  addr7/1 -> dout/1

== system rfsoc4x2_ospfb_128/pfb_fir_real9/adder_1_7 ==
  sync : Inport
  din1 : Inport  Port=2
  din2 : Inport  Port=3
  din3 : Inport  Port=4
  din4 : Inport  Port=5
  din5 : Inport  Port=6
  din6 : Inport  Port=7
  din7 : Inport  Port=8
  din8 : Inport  Port=9
  addr{1..4} (4 alike) : xbsIndex_r4/AddSub  mode=Addition  use_carryin=off  use_carryout=off  en=off  latency=1  precision=User Defined  arith_type="Signed  (2's comp)"  n_bits=32  bin_pt=30  quantization=Truncate  overflow=Wrap  use_behavioral_HDL=on  hw_selection=Fabric  pipelined=on  use_rpm=on  dbl_ovrd=off  block_type=addsub
  addr5 : xbsIndex_r4/AddSub  mode=Addition  use_carryin=off  use_carryout=off  en=off  latency=1  precision=User Defined  arith_type="Signed  (2's comp)"  n_bits=32  bin_pt=30  quantization=Truncate  overflow=Wrap  use_behavioral_HDL=off  hw_selection=Fabric  pipelined=on  use_rpm=on  dbl_ovrd=off  block_type=addsub
  addr6 : xbsIndex_r4/AddSub  mode=Addition  use_carryin=off  use_carryout=off  en=off  latency=1  precision=User Defined  arith_type="Signed  (2's comp)"  n_bits=32  bin_pt=30  quantization=Truncate  overflow=Wrap  use_behavioral_HDL=off  hw_selection=Fabric  pipelined=on  use_rpm=on  dbl_ovrd=off  block_type=addsub
  addr7 : xbsIndex_r4/AddSub  mode=Addition  use_carryin=off  use_carryout=off  en=off  latency=1  precision=User Defined  arith_type="Signed  (2's comp)"  n_bits=32  bin_pt=30  quantization=Truncate  overflow=Wrap  use_behavioral_HDL=off  hw_selection=Fabric  pipelined=on  use_rpm=on  dbl_ovrd=off  block_type=addsub
  sync_delay : xbsIndex_r4/Delay  rst=off  infoeditControl=Selection of Reset will increase slice count due to use of real FFs and instead of SRLs  en=off  latency=3  reg_retiming=on  dbl_ovrd=off  block_type=delay
      settings: block_version=11.4
  sync_out : Outport  VectorParamsAs1DForOutWhenUnconnected=off
  dout : Outport  Port=2  VectorParamsAs1DForOutWhenUnconnected=off
  wires:
  sync/1 -> sync_delay/1
  sync_delay/1 -> sync_out/1
  din1/1 -> addr1/1
  din2/1 -> addr1/2
  din3/1 -> addr2/1
  din4/1 -> addr2/2
  din5/1 -> addr3/1
  din6/1 -> addr3/2
  din7/1 -> addr4/1
  din8/1 -> addr4/2
  addr1/1 -> addr5/1
  addr2/1 -> addr5/2
  addr3/1 -> addr6/1
  addr4/1 -> addr6/2
  addr5/1 -> addr7/1
  addr6/1 -> addr7/2
  addr7/1 -> dout/1

== system rfsoc4x2_ospfb_128/pfb_fir_real9/adder_1_8 ==
  sync : Inport
  din1 : Inport  Port=2
  din2 : Inport  Port=3
  din3 : Inport  Port=4
  din4 : Inport  Port=5
  din5 : Inport  Port=6
  din6 : Inport  Port=7
  din7 : Inport  Port=8
  din8 : Inport  Port=9
  addr{1..4} (4 alike) : xbsIndex_r4/AddSub  mode=Addition  use_carryin=off  use_carryout=off  en=off  latency=1  precision=User Defined  arith_type="Signed  (2's comp)"  n_bits=32  bin_pt=30  quantization=Truncate  overflow=Wrap  use_behavioral_HDL=on  hw_selection=Fabric  pipelined=on  use_rpm=on  dbl_ovrd=off  block_type=addsub
  addr5 : xbsIndex_r4/AddSub  mode=Addition  use_carryin=off  use_carryout=off  en=off  latency=1  precision=User Defined  arith_type="Signed  (2's comp)"  n_bits=32  bin_pt=30  quantization=Truncate  overflow=Wrap  use_behavioral_HDL=off  hw_selection=Fabric  pipelined=on  use_rpm=on  dbl_ovrd=off  block_type=addsub
  addr6 : xbsIndex_r4/AddSub  mode=Addition  use_carryin=off  use_carryout=off  en=off  latency=1  precision=User Defined  arith_type="Signed  (2's comp)"  n_bits=32  bin_pt=30  quantization=Truncate  overflow=Wrap  use_behavioral_HDL=off  hw_selection=Fabric  pipelined=on  use_rpm=on  dbl_ovrd=off  block_type=addsub
  addr7 : xbsIndex_r4/AddSub  mode=Addition  use_carryin=off  use_carryout=off  en=off  latency=1  precision=User Defined  arith_type="Signed  (2's comp)"  n_bits=32  bin_pt=30  quantization=Truncate  overflow=Wrap  use_behavioral_HDL=off  hw_selection=Fabric  pipelined=on  use_rpm=on  dbl_ovrd=off  block_type=addsub
  sync_delay : xbsIndex_r4/Delay  rst=off  infoeditControl=Selection of Reset will increase slice count due to use of real FFs and instead of SRLs  en=off  latency=3  reg_retiming=on  dbl_ovrd=off  block_type=delay
      settings: block_version=11.4
  sync_out : Outport  VectorParamsAs1DForOutWhenUnconnected=off
  dout : Outport  Port=2  VectorParamsAs1DForOutWhenUnconnected=off
  wires:
  sync/1 -> sync_delay/1
  sync_delay/1 -> sync_out/1
  din1/1 -> addr1/1
  din2/1 -> addr1/2
  din3/1 -> addr2/1
  din4/1 -> addr2/2
  din5/1 -> addr3/1
  din6/1 -> addr3/2
  din7/1 -> addr4/1
  din8/1 -> addr4/2
  addr1/1 -> addr5/1
  addr2/1 -> addr5/2
  addr3/1 -> addr6/1
  addr4/1 -> addr6/2
  addr5/1 -> addr7/1
  addr6/1 -> addr7/2
  addr7/1 -> dout/1

== system rfsoc4x2_ospfb_128/pfb_fir_real9/adder_1_9 ==
  sync : Inport
  din1 : Inport  Port=2
  din2 : Inport  Port=3
  din3 : Inport  Port=4
  din4 : Inport  Port=5
  din5 : Inport  Port=6
  din6 : Inport  Port=7
  din7 : Inport  Port=8
  din8 : Inport  Port=9
  addr{1..4} (4 alike) : xbsIndex_r4/AddSub  mode=Addition  use_carryin=off  use_carryout=off  en=off  latency=1  precision=User Defined  arith_type="Signed  (2's comp)"  n_bits=32  bin_pt=30  quantization=Truncate  overflow=Wrap  use_behavioral_HDL=on  hw_selection=Fabric  pipelined=on  use_rpm=on  dbl_ovrd=off  block_type=addsub
  addr5 : xbsIndex_r4/AddSub  mode=Addition  use_carryin=off  use_carryout=off  en=off  latency=1  precision=User Defined  arith_type="Signed  (2's comp)"  n_bits=32  bin_pt=30  quantization=Truncate  overflow=Wrap  use_behavioral_HDL=off  hw_selection=Fabric  pipelined=on  use_rpm=on  dbl_ovrd=off  block_type=addsub
  addr6 : xbsIndex_r4/AddSub  mode=Addition  use_carryin=off  use_carryout=off  en=off  latency=1  precision=User Defined  arith_type="Signed  (2's comp)"  n_bits=32  bin_pt=30  quantization=Truncate  overflow=Wrap  use_behavioral_HDL=off  hw_selection=Fabric  pipelined=on  use_rpm=on  dbl_ovrd=off  block_type=addsub
  addr7 : xbsIndex_r4/AddSub  mode=Addition  use_carryin=off  use_carryout=off  en=off  latency=1  precision=User Defined  arith_type="Signed  (2's comp)"  n_bits=32  bin_pt=30  quantization=Truncate  overflow=Wrap  use_behavioral_HDL=off  hw_selection=Fabric  pipelined=on  use_rpm=on  dbl_ovrd=off  block_type=addsub
  sync_delay : xbsIndex_r4/Delay  rst=off  infoeditControl=Selection of Reset will increase slice count due to use of real FFs and instead of SRLs  en=off  latency=3  reg_retiming=on  dbl_ovrd=off  block_type=delay
      settings: block_version=11.4
  sync_out : Outport  VectorParamsAs1DForOutWhenUnconnected=off
  dout : Outport  Port=2  VectorParamsAs1DForOutWhenUnconnected=off
  wires:
  sync/1 -> sync_delay/1
  sync_delay/1 -> sync_out/1
  din1/1 -> addr1/1
  din2/1 -> addr1/2
  din3/1 -> addr2/1
  din4/1 -> addr2/2
  din5/1 -> addr3/1
  din6/1 -> addr3/2
  din7/1 -> addr4/1
  din8/1 -> addr4/2
  addr1/1 -> addr5/1
  addr2/1 -> addr5/2
  addr3/1 -> addr6/1
  addr4/1 -> addr6/2
  addr5/1 -> addr7/1
  addr6/1 -> addr7/2
  addr7/1 -> dout/1

== system rfsoc4x2_ospfb_128/pfb_fir_real9/edge_detect8 ==
  in : Inport
  Delay : xbsIndex_r4/Delay  rst=off  infoeditControl=Selection of Reset will increase slice count due to use of real FFs and instead of SRLs  en=off  latency=1  reg_retiming=off  dbl_ovrd=off  block_type=delay
      settings: xl_area=[0, 0, 0, 0, 0, 0, 0]
  Inverter : xbsIndex_r4/Inverter  en=off  latency=0  dbl_ovrd=off  block_type=inv
      settings: xl_area=[0, 0, 0, 0, 0, 0, 0]
  edge_op : xbsIndex_r4/Logical  logical_function=AND  inputs=2  en=off  latency=0  precision=Full  arith_type=Unsigned  n_bits=8  bin_pt=2  align_bp=on  dbl_ovrd=off  block_type=logical
      settings: xl_area=[0, 0, 0, 0, 0, 0, 0]
  out : Outport  VectorParamsAs1DForOutWhenUnconnected=off
  wires:
  Delay/1 -> edge_op/2
  in/1 -> Delay/1, Inverter/1
  edge_op/1 -> out/1
  Inverter/1 -> edge_op/1
